simulink model "Ex5_LS3"  (R2025a)
settings: Solver=ode45  StartTime=0.0  StopTime=5  MaxStep=0.1  MinStep=0.1  RelTol=1e-3  EnableMultiTasking=on
values from neighbouring files (symbols this model uses):
  Beff = [50 50 50]    [Ex5_LS3_code.m]
  F = 5    [Ex5_LS3_code.m]
  Jeff = [14 14 14]    [Ex5_LS3_code.m]
  K = 2750    [Ex5_LS3_code.m]
  Kd = [(2*wn*Jeff(1) - Beff(1))/K (2*wn*Jeff(2) - Beff(2))/K (2*wn*Jeff(3) - Beff(3))/K]    [Ex5_LS3_code.m]
  Kp = [(Jeff(1)*wn*wn)/K (Jeff(2)*wn*wn)/K (Jeff(3)*wn*wn)/K]    [Ex5_LS3_code.m]
  L = [0.5; 0.3]    [Ex5_LS3_code.m]
  m = [4.6; 2.3; 1.0]    [Ex5_LS3_code.m]
  N = 3    [Ex5_LS3_code.m]
  r = 1/100    (= 0.01)    [Ex5_LS3_code.m]
undefined symbols (not defined in the file or in its folder): ThetaA_0, W_0, XdotC0
libraries: slpidlib x1
settings Model: Creator=aluno  LastModifiedBy=Gabriel Toledo
settings SolverCC: InitialStep=0.1  AlgebraicLoopSolver=TrustRegion
settings DataIOCC: LimitDataPoints=on  SaveFormat=Array  ReturnWorkspaceOutputs=off
settings OptimizationCC: LifeSpan=inf
settings DebuggingCC: SolverPrmCheckMsg=warning  UnconnectedInputMsg=warning  UnconnectedOutputMsg=warning  UnconnectedLineMsg=warning  SFUnexpectedBacktrackingDiag=warning  SFNoUnconditionalDefaultTransitionDiag=warning  SFExecutionAtInitializationDiag=none  ArithmeticOperatorsInVariantConditions=warning
settings HardwareCC: ProdBitPerPointer=32.0  ProdBitPerSizeT=32.0  ProdBitPerPtrDiffT=32.0  ProdLargestAtomicFloat=None  ProdIntDivRoundTo=Undefined  ProdEndianess=Unspecified  ProdWordSize=32.0  ProdHWDeviceType=32-bit Generic
settings ModelReferenceCC: PropagateSignalLabelsOutOfModel=off
settings SFSimCC: SimUseLocalCustomCode=off  CustomCodeUndefinedFunction=UseInterfaceOnly
settings RTWCC: RTWUseLocalCustomCode=off  GPUComputeCapability=3.5
settings CodeAppCC: StateflowObjectComments=on
settings GRTTargetCC: TargetLangStandard=C89/C90 (ANSI)
settings ConfigComp: CovMetricSettings=dw  CovSaveCumulativeToWorkspaceVar=on  CovSaveSingleToWorkspaceVar=on  CovExternalEMLEnable=off  CovSFcnEnable=off

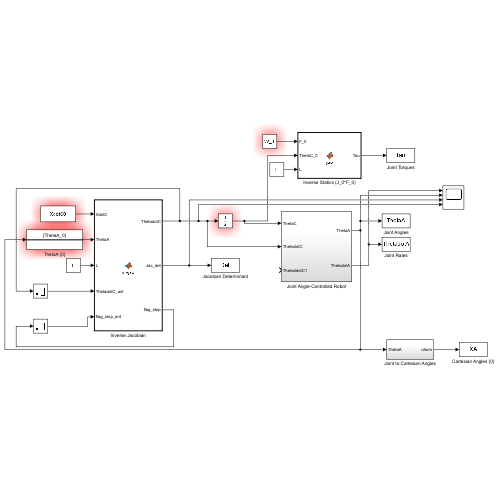
[thumbnail: Simulink's stored preview of the top-level diagram]
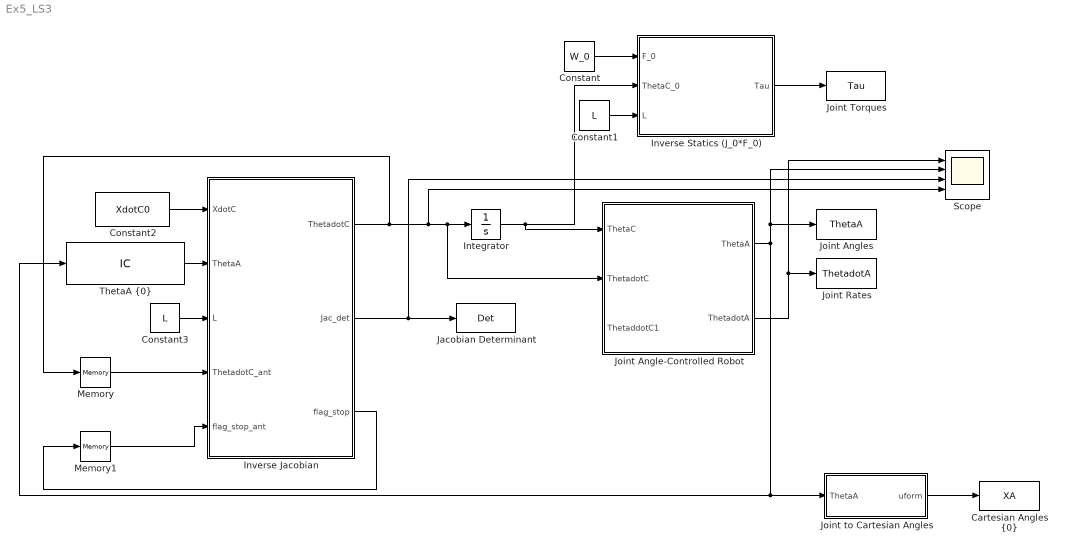
== system Ex5_LS3 ==
  "Cartesian Angles {0}" : ToWorkspace  VariableName=XA  SaveFormat=Timeseries  SampleTime=-1
  Constant : Constant  Value=W_0
  Constant1 : Constant  Value=L
  Constant2 : Constant  Value=XdotC0
  Constant3 : Constant  Value=L
  Integrator : Integrator  InitialCondition=ThetaA_0
  Inverse Jacobian : MATLAB Function  TreatAsAtomicUnit=on
  Inverse Statics (J_0*F_0) : MATLAB Function  TreatAsAtomicUnit=on
  Jacobian Determinant : ToWorkspace  VariableName=Det  SaveFormat=Timeseries  SampleTime=-1
  Joint Angle-Controlled Robot : Subsystem
  Joint Angles : ToWorkspace  VariableName=ThetaA  SaveFormat=Timeseries  SampleTime=-1
  Joint Rates : ToWorkspace  VariableName=ThetadotA  SaveFormat=Timeseries  SampleTime=-1
  Joint Torques : ToWorkspace  VariableName=Tau  SaveFormat=Timeseries  SampleTime=-1
  Joint to Cartesian Angles : Subsystem
  Memory : Memory
  Memory1 : Memory
  Scope : Scope  NumInputPorts=4
      settings: ActiveDisplayYMinimum=-5  ActiveDisplayYMaximum=5  DataLoggingSaveFormat=Array
  "ThetaA {0}" : InitialCondition  Value=ThetaA_0
  wires:
  Constant3/1 -> Inverse Jacobian/3(L)
  Constant2/1 -> Inverse Jacobian/1(XdotC)
  Inverse Jacobian/1(ThetadotC) -> Memory/1, Scope/4, Joint Angle-Controlled Robot/2(ThetadotC), Integrator/1
  Inverse Jacobian/3(flag_stop) -> Memory1/1
  Inverse Jacobian/2(Jac_det) -> Scope/3, Jacobian Determinant/1
  "ThetaA {0}"/1 -> Inverse Jacobian/2(ThetaA)
  Integrator/1 -> Joint Angle-Controlled Robot/1(ThetaC), Inverse Statics (J_0*F_0)/2(ThetaC_0)
  Inverse Statics (J_0*F_0)/1(Tau) -> Joint Torques/1
  Joint Angle-Controlled Robot/2(ThetadotA) -> Scope/1, Joint Rates/1
  Joint Angle-Controlled Robot/1(ThetaA) -> Scope/2, Joint Angles/1, Joint to Cartesian Angles/1(ThetaA), "ThetaA {0}"/1
  Joint to Cartesian Angles/1(uform) -> "Cartesian Angles {0}"/1
  Constant/1 -> Inverse Statics (J_0*F_0)/1(F_0)
  Constant1/1 -> Inverse Statics (J_0*F_0)/3(L)
  Memory/1 -> Inverse Jacobian/4(ThetadotC_ant)
  Memory1/1 -> Inverse Jacobian/5(flag_stop_ant)

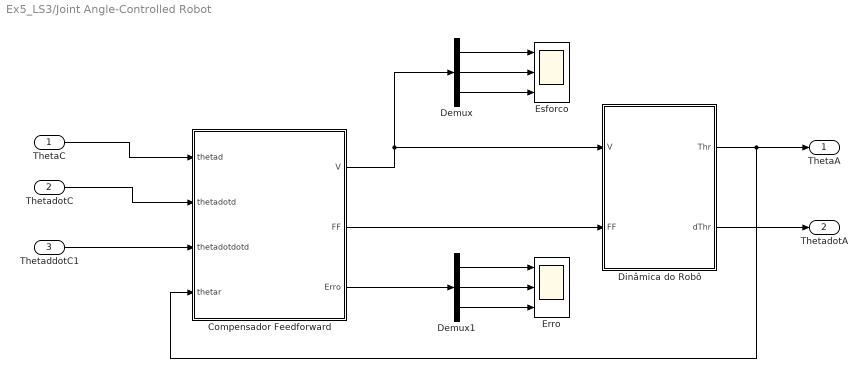
== system Ex5_LS3/Joint Angle-Controlled Robot ==
  ThetaC : Inport
  ThetadotC : Inport  Port=2
  ThetaddotC1 : Inport  Port=3
  Compensador Feedforward : Subsystem
  Demux : Demux  Outputs=3
  Demux1 : Demux  Outputs=3
  Dinâmica do Robô : Subsystem
  Erro : Scope  NumInputPorts=3
      settings: ActiveDisplayYMinimum=-0.0091697119544363326  ActiveDisplayYMaximum=0.15631954074254673  DataLoggingVariableName=Erro
  Esforco : Scope  NumInputPorts=3
      settings: ActiveDisplayYMinimum=-4861.2652  ActiveDisplayYMaximum=4798.38005  DataLoggingVariableName=Esforco
  ThetaA : Outport
  ThetadotA : Outport  Port=2
  wires:
  Demux/3 -> Esforco/3
  Dinâmica do Robô/1(Thr) -> ThetaA/1, Compensador Feedforward/4(thetar)
  Dinâmica do Robô/2(dThr) -> ThetadotA/1
  Demux1/3 -> Erro/3
  Compensador Feedforward/1(V) -> Demux/1, Dinâmica do Robô/1(V)
  Demux/1 -> Esforco/1
  Compensador Feedforward/3(Erro) -> Demux1/1
  Compensador Feedforward/2(FF) -> Dinâmica do Robô/2(FF)
  Demux1/1 -> Erro/1
  Demux1/2 -> Erro/2
  Demux/2 -> Esforco/2
  ThetaC/1 -> Compensador Feedforward/1(thetad)
  ThetadotC/1 -> Compensador Feedforward/2(thetadotd)
  ThetaddotC1/1 -> Compensador Feedforward/3(thetadotdotd)

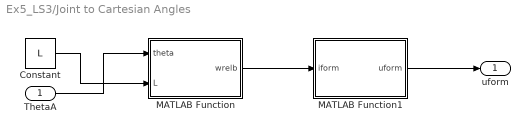
== system Ex5_LS3/Joint to Cartesian Angles ==
  ThetaA : Inport
  Constant : Constant  Value=L
  MATLAB Function : MATLAB Function  TreatAsAtomicUnit=on
  MATLAB Function1 : MATLAB Function  TreatAsAtomicUnit=on
  uform : Outport
  wires:
  ThetaA/1 -> MATLAB Function/1(theta)
  Constant/1 -> MATLAB Function/2(L)
  MATLAB Function/1(wrelb) -> MATLAB Function1/1(iform)
  MATLAB Function1/1(uform) -> uform/1

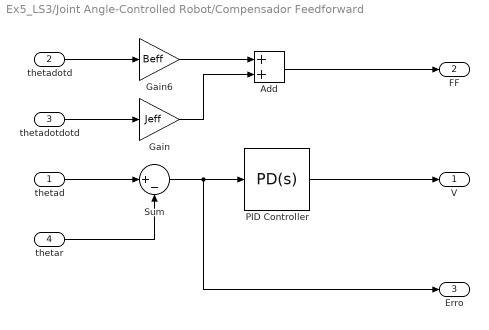
== system Ex5_LS3/Joint Angle-Controlled Robot/Compensador Feedforward ==
  thetad : Inport
  thetadotd : Inport  Port=2
  thetadotdotd : Inport  Port=3
  thetar : Inport  Port=4
  Add : Sum
  Gain : Gain  Gain=Jeff
  Gain6 : Gain  Gain=Beff
  PID Controller : slpidlib/PID Controller  Controller=PD  Form=Parallel  TimeDomain=Continuous-time  UseExternalTs=off  SampleTime=-1  IntegratorMethod=Forward Euler  FilterMethod=Forward Euler  ControllerParametersSource=internal  P=Kp  I=1  UseKiTs=off  D=Kd  UseExternalDerivativeSource=off  N=N  UseFilter=on  TunerSelectOption=Transfer Function Based (PID Tuner App)  InitialConditionSource=internal  InitialConditionForIntegrator=0  InitialConditionForFilter=0  DifferentiatorICPrevScaledInput=0  ExternalReset=none  TrackingMode=off  Kt=1  LimitOutput=off  SatLimitsSource=internal  UpperSaturationLimit=inf  LowerSaturationLimit=-inf  LinearizeAsGain=on  AntiWindupMode=none  Kb=1  LimitIntegrator=off  UpperIntegratorSaturationLimit=inf  LowerIntegratorSaturationLimit=-inf  POutMin=[]  POutMax=[]  IOutMin=[]  IOutMax=[]  DOutMin=[]  DOutMax=[]  NOutMin=[]  NOutMax=[]  SumOutMin=[]  SumOutMax=[]  SaturationOutMin=[]  SaturationOutMax=[]  PParamMin=[]  PParamMax=[]  IParamMin=[]  IParamMax=[]  DParamMin=[]  DParamMax=[]  NParamMin=[]  NParamMax=[]  KbParamMin=[]  KbParamMax=[]  KtParamMin=[]  KtParamMax=[]  KbOutMin=[]  KbOutMax=[]  KtOutMin=[]  KtOutMax=[]  IntegratorOutMin=[]  IntegratorOutMax=[]  FilterOutMin=[]  FilterOutMax=[]  SumI1OutMin=[]  SumI1OutMax=[]  SumI2OutMin=[]  SumI2OutMax=[]  SumI3OutMin=[]  SumI3OutMax=[]  SumI4OutMin=[]  SumI4OutMax=[]  SumDOutMin=[]  SumDOutMax=[]  DifferentiatorOutMin=[]  DifferentiatorOutMax=[]  FilterDiffOutCoefMin=[]  FilterDiffOutCoefMax=[]  ReciprocalOutMin=[]  ReciprocalOutMax=[]  SumDenOutMin=[]  SumDenOutMax=[]  SumNumOutMin=[]  SumNumOutMax=[]  DivideOutMin=[]  DivideOutMax=[]  UdiffTsProdOutMin=[]  UdiffTsProdOutMax=[]  NTsProdOutMin=[]  NTsProdOutMax=[]  UintegralTsProdOutMin=[]  UintegralTsProdOutMax=[]  UngainTsProdOutMin=[]  UngainTsProdOutMax=[]  ClampingZeroOutDataTypeStr=Inherit: Inherit via back propagation  ClampingZeroOutMin=[]  ClampingZeroOutMax=[]  FilterDenConstantOutDataTypeStr=Inherit: Inherit via back propagation  FilterDenConstantOutMin=[]  FilterDenConstantOutMax=[]  PCopyOutDataTypeStr=Inherit: Inherit via back propagation  PCopyOutMin=[]  PCopyOutMax=[]  NCopyOutDataTypeStr=Inherit: Inherit via back propagation  NCopyOutMin=[]  NCopyOutMax=[]  IntegratorContinuousStateAttributes=''  IntegratorStateMustResolveToSignalObject=off  IntegratorRTWStateStorageClass=Auto  FilterContinuousStateAttributes=''  FilterStateMustResolveToSignalObject=off  FilterRTWStateStorageClass=Auto  ParallelPVariant=InternalParameters  IdealPVariant=Disabled  IVariant=Disabled  DVariant=InternalParameters  IntegratorVariant=Disabled  SatVariant=Disabled  AWVariant=Disabled  PCopyVariant=Disabled  TRVariant=Disabled  FdbkBlocksVariant=Forward  IdealPFdbkVariant=Disabled  SatFdbkVariant=Disabled  DerivativeFilterVariant=ContFilter  NVariant=InternalParameters  NCopyVariant=Disabled  FilterICVariant=InternalICsFilter  IntegratorICVariant=Disabled  ExternalResetVariant=Disabled  TRSumVariant=Passthrough  SumFdbkVariant=Disabled  SumVariant=Sum_PD  TsampFilterVariant=InternalTs  TsampNgainVariant=Passthrough  TsampIntegralVariant=Disabled_SignalSpec  ExternalSaturationOutDataTypeStr=Inherit: Same as second input  DerivativeSourceVariant=ErrorSignal  PreIntVariant=InternalPreInt
  Sum : Sum  Inputs=|+-
  V : Outport
  FF : Outport  Port=2
  Erro : Outport  Port=3
  wires:
  thetadotd/1 -> Gain6/1
  Gain6/1 -> Add/1
  Gain/1 -> Add/2
  thetadotdotd/1 -> Gain/1
  thetad/1 -> Sum/1
  thetar/1 -> Sum/2
  Sum/1 -> PID Controller/1, Erro/1
  Add/1 -> FF/1
  PID Controller/1 -> V/1

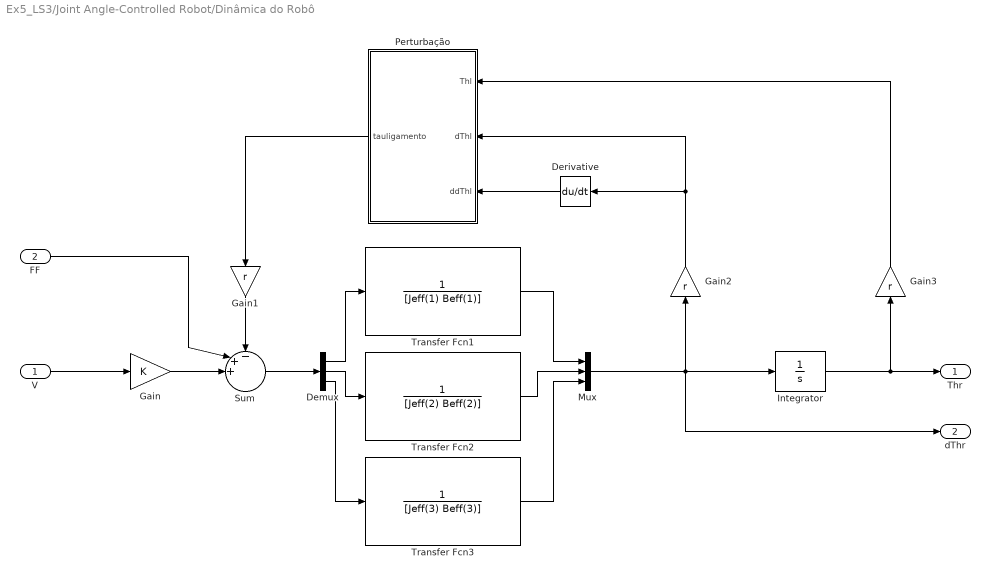
== system Ex5_LS3/Joint Angle-Controlled Robot/Dinâmica do Robô ==
  V : Inport
  FF : Inport  Port=2
  Demux : Demux  Outputs=3
  Derivative : Derivative
  Gain : Gain  Gain=K
  Gain1 : Gain  Gain=r
  Gain2 : Gain  Gain=r
  Gain3 : Gain  Gain=r
  Integrator : Integrator
  Mux : Mux  Inputs=3
  Perturbação : Subsystem
  Sum : Sum  Inputs=-++||
  Transfer Fcn1 : TransferFcn  Denominator=[Jeff(1) Beff(1)]
  Transfer Fcn2 : TransferFcn  Denominator=[Jeff(2) Beff(2)]
  Transfer Fcn3 : TransferFcn  Denominator=[Jeff(3) Beff(3)]
  Thr : Outport
  dThr : Outport  Port=2
  wires:
  Integrator/1 -> Gain3/1, Thr/1
  Gain2/1 -> Perturbação/2(dThl), Derivative/1
  Derivative/1 -> Perturbação/3(ddThl)
  Perturbação/1(tauligamento) -> Gain1/1
  Gain3/1 -> Perturbação/1(Thl)
  V/1 -> Gain/1
  Gain1/1 -> Sum/1
  Gain/1 -> Sum/3
  FF/1 -> Sum/2
  Sum/1 -> Demux/1
  Demux/1 -> Transfer Fcn1/1
  Mux/1 -> dThr/1, Gain2/1, Integrator/1
  Transfer Fcn1/1 -> Mux/1
  Transfer Fcn3/1 -> Mux/3
  Transfer Fcn2/1 -> Mux/2
  Demux/2 -> Transfer Fcn2/1
  Demux/3 -> Transfer Fcn3/1

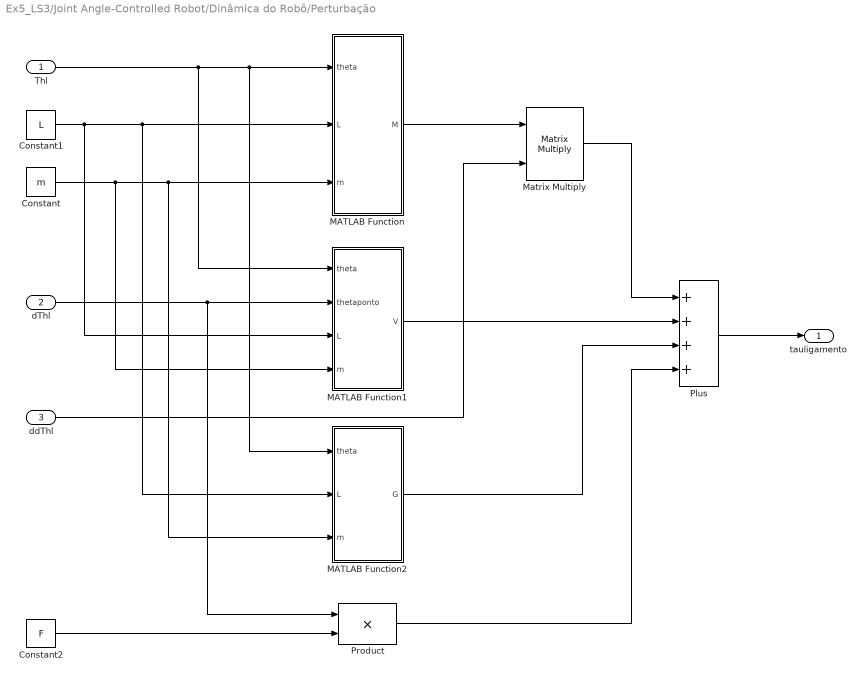
== system Ex5_LS3/Joint Angle-Controlled Robot/Dinâmica do Robô/Perturbação ==
  Thl : Inport
  dThl : Inport  Port=2
  ddThl : Inport  Port=3
  Constant : Constant  Value=m
  Constant1 : Constant  Value=L
  Constant2 : Constant  Value=F
  MATLAB Function : MATLAB Function  TreatAsAtomicUnit=on
  MATLAB Function1 : MATLAB Function  TreatAsAtomicUnit=on
  MATLAB Function2 : MATLAB Function  TreatAsAtomicUnit=on
  Matrix Multiply : Product  Multiplication=Matrix(*)
  Plus : Sum  Inputs=++++
  Product : Product
  tauligamento : Outport
  wires:
  Constant/1 -> MATLAB Function1/4(m), MATLAB Function2/3(m), MATLAB Function/3(m)
  Constant1/1 -> MATLAB Function1/3(L), MATLAB Function2/2(L), MATLAB Function/2(L)
  Thl/1 -> MATLAB Function1/1(theta), MATLAB Function2/1(theta), MATLAB Function/1(theta)
  dThl/1 -> Product/1, MATLAB Function1/2(thetaponto)
  Plus/1 -> tauligamento/1
  MATLAB Function1/1(V) -> Plus/2
  MATLAB Function2/1(G) -> Plus/3
  Constant2/1 -> Product/2
  Product/1 -> Plus/4
  MATLAB Function/1(M) -> Matrix Multiply/1
  ddThl/1 -> Matrix Multiply/2
  Matrix Multiply/1 -> Plus/1

== matlab function Ex5_LS3/Inverse Statics (J_0*F_0) ==
  data: F_0 input; Tau output; ThetaC_0 input; L input
function Tau = jac(F_0, ThetaC_0, L)
%#codegen

J0 = [ -L(1)*sin(ThetaA(1)) - L(2)*sin(ThetaA(1)+ThetaA(2)), -L(2)*sin(ThetaA(1)+ThetaA(2)), 0;
       -L(1)*cos(ThetaA(1)) + L(2)*cos(ThetaA(1)+ThetaA(2)),  L(2)*cos(ThetaA(1)+ThetaA(2)), 0;
       1,                                                     1,                            1];

Tau = J0'*F_0;

end

== matlab function Ex5_LS3/Inverse Jacobian ==
  data: XdotC input; ThetadotC output; ThetaA input; L input; ThetadotC_ant input; flag_stop_ant input; Jac_det output; flag_stop output
function [ThetadotC, Jac_det, flag_stop]= invjac(XdotC, ThetaA, L, ThetadotC_ant, flag_stop_ant)
%#codegen

tolerance = 1e-6;

J0 = [ -L(1)*sind(ThetaA(1)) - L(2)*sind(ThetaA(1)+ThetaA(2)), -L(2)*sind(ThetaA(1)+ThetaA(2)), 0;
        L(1)*cosd(ThetaA(1)) + L(2)*cosd(ThetaA(1)+ThetaA(2)),  L(2)*cosd(ThetaA(1)+ThetaA(2)), 0;
       1,                                                       1,                             1];
   
Jac_det = det(J0);

flag_stop = flag_stop_ant;

if abs(Jac_det) < tolerance
    ThetadotC = ThetadotC_ant;
else
    inv_JO = J0^-1;
    ThetadotC = inv_JO*XdotC;
end

end

== matlab function Ex5_LS3/Joint to Cartesian Angles/MATLAB Function ==
  data: theta input; wrelb output; L input
%% Function
function wrelb = kin(theta, L)
%% Main Calculations

    Theta = theta(1) + theta(2) + theta(3);
    T = [cos(Theta)   -sin(Theta) 0 L(1)*cos(theta(1)) + L(2)*cos(theta(1) + theta(2));
         sin(Theta)    cos(Theta) 0 L(1)*sin(theta(1)) + L(2)*sin(theta(1) + theta(2));
         0              0           1 0;
         0              0           0 1];

%% Output Data

    wrelb = T;
    
end

== matlab function Ex5_LS3/Joint to Cartesian Angles/MATLAB Function1 ==
  data: iform input; uform output
%% Function
function uform = itou(iform)

%% Validity


%% Main Calculations

    theta = atan2(iform(2, 1),iform(1, 1));
    
    T = [iform(1, 4) iform(2, 4) theta];

%% Output Data

    uform = T;
    
end

== matlab function Ex5_LS3/Joint Angle-Controlled Robot/Dinâmica do Robô/Perturbação/MATLAB Function ==
  data: theta input; M output; L input; m input
function M = matriz_m(theta, L, m)

    M = [0,                                                 (m(2)+m(3))*(L(2)^2+L(1)*L(2))*cos(theta(3))+0.1,      0.1;
         (m(2)+m(3))*(L(2)^2+L(1)*L(2)*cos(theta(2)))+0.1,  0,                                                     0.1;
         0.1,                                               0.1,                                                   0];

== matlab function Ex5_LS3/Joint Angle-Controlled Robot/Dinâmica do Robô/Perturbação/MATLAB Function1 ==
  data: theta input; thetaponto input; V output; L input; m input
function V = matriz_v(theta, thetaponto, L, m)
    
    V = [-(m(2)+m(3))*L(1)*L(2)*sin(theta(2))*(thetaponto(2)^2+thetaponto(1)*thetaponto(2));
         (m(2)+m(3))*L(1)*L(2)*sin(theta(2))*thetaponto(1)^2;
         0];

== matlab function Ex5_LS3/Joint Angle-Controlled Robot/Dinâmica do Robô/Perturbação/MATLAB Function2 ==
  data: theta input; G output; L input; m input
function G = matriz_g(theta, L, m)
 
    G = [(m(1)+m(2)+m(3))*L(1)*cos(theta(1))+(m(2)+m(3))*(L(2)*cos(theta(1)+theta(2)));
         (m(2)+m(3))*(L(2)*cos(theta(1)+theta(2)));
         0];
